simulink model "KFFA_LADRC_Quadrotor"  (R2026a)
settings: Solver=ode1  StopTime=15.0  FixedStep=0.001
InitFcn:
  | setup;
undefined symbols (not defined in the file or in its folder): b0_z, g, Ix, Iy, Iz, Kf, l0, M, Q_kf, R_kf, wc_z, wo_z, z2
settings Model: Creator=thanu  LastModifiedBy=thanu
settings DebuggingCC: UnderSpecifiedDimensionMsg=warning

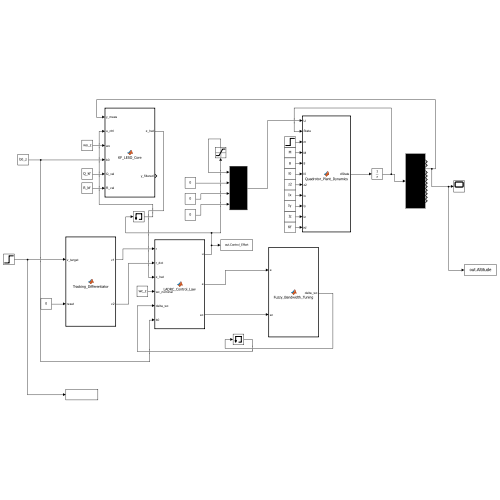
[thumbnail: Simulink's stored preview of the top-level diagram]
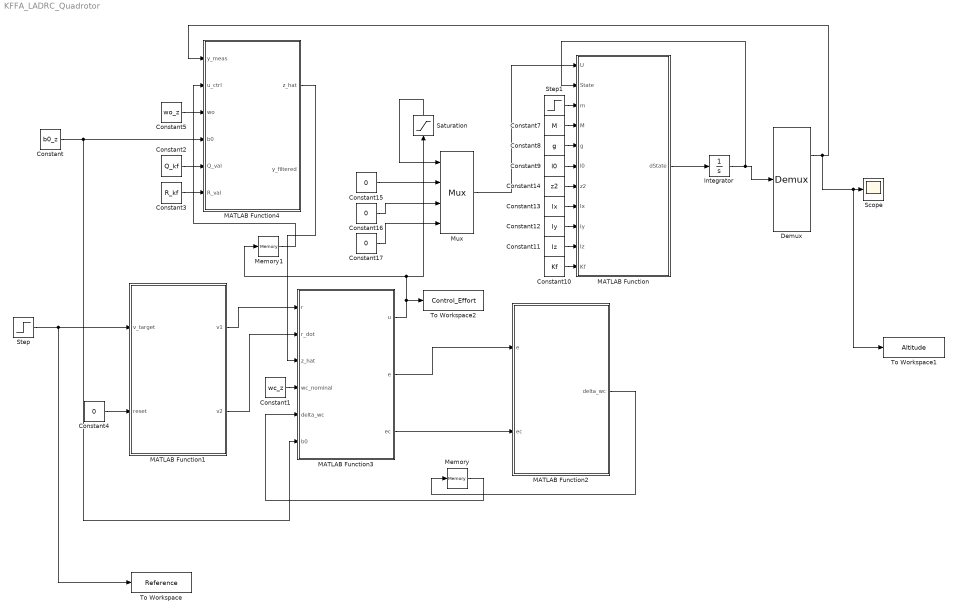
== system KFFA_LADRC_Quadrotor ==
  Constant : Constant  Value=b0_z
  Constant1 : Constant  Value=wc_z
  Constant10 : Constant  Value=Kf
  Constant11 : Constant  Value=Iz
  Constant12 : Constant  Value=Iy
  Constant13 : Constant  Value=Ix
  Constant14 : Constant  Value=z2
  Constant{4,15..17} (4 alike) : Constant  Value=0
  Constant2 : Constant  Value=Q_kf
  Constant3 : Constant  Value=R_kf
  Constant5 : Constant  Value=wo_z
  Constant7 : Constant  Value=M
  Constant8 : Constant  Value=g
  Constant9 : Constant  Value=l0
  Demux : Demux  Outputs=12
  Integrator : Integrator  InitialCondition=zeros(12,1)
  MATLAB Function : MATLAB Function  TreatAsAtomicUnit=on
  MATLAB Function1 : MATLAB Function  TreatAsAtomicUnit=on
  MATLAB Function2 : MATLAB Function  TreatAsAtomicUnit=on
  MATLAB Function3 : MATLAB Function  TreatAsAtomicUnit=on
  MATLAB Function4 : MATLAB Function  TreatAsAtomicUnit=on
  Memory : Memory
  Memory1 : Memory
  Mux : Mux
  Saturation : Saturate  UpperLimit=650  LowerLimit=0
  Scope : Scope
      settings: ActiveDisplayYMinimum=3.8784295191578879  ActiveDisplayYMaximum=5.8241533888840671
  Step : Step  FinalValue=5  SampleTime=0
  Step1 : Step  Time=5  FinalValue=m_payload_val  SampleTime=0
  To Workspace : ToWorkspace  VariableName=Reference  SampleTime=-1
  To Workspace1 : ToWorkspace  VariableName=Altitude  SampleTime=-1
  To Workspace2 : ToWorkspace  VariableName=Control_Effort  SampleTime=-1
  wires:
  Step/1 -> To Workspace/1, MATLAB Function1/1(v_target)
  Constant4/1 -> MATLAB Function1/2(reset)
  MATLAB Function1/1(v1) -> MATLAB Function3/1(r)
  MATLAB Function1/2(v2) -> MATLAB Function3/2(r_dot)
  MATLAB Function3/2(e) -> MATLAB Function2/1(e)
  MATLAB Function3/3(ec) -> MATLAB Function2/2(ec)
  MATLAB Function4/1(z_hat) -> MATLAB Function3/3(z_hat)
  Mux/1 -> MATLAB Function/1(U)
  MATLAB Function/1(dState) -> Integrator/1
  Integrator/1 -> Demux/1, MATLAB Function/2(State)
  Demux/3 -> To Workspace1/1, Scope/1, MATLAB Function4/1(y_meas)
  Constant1/1 -> MATLAB Function3/4(wc_nominal)
  Constant3/1 -> MATLAB Function4/6(R_val)
  Constant2/1 -> MATLAB Function4/5(Q_val)
  Step1/1 -> MATLAB Function/3(m)
  Constant7/1 -> MATLAB Function/4(M)
  Constant8/1 -> MATLAB Function/5(g)
  Constant9/1 -> MATLAB Function/6(l0)
  Constant10/1 -> MATLAB Function/11(Kf)
  Constant11/1 -> MATLAB Function/10(Iz)
  Constant12/1 -> MATLAB Function/9(Iy)
  Constant13/1 -> MATLAB Function/8(Ix)
  Constant14/1 -> MATLAB Function/7(z2)
  Constant15/1 -> Mux/2
  Constant16/1 -> Mux/3
  Constant17/1 -> Mux/4
  Constant/1 -> MATLAB Function3/6(b0), MATLAB Function4/4(b0)
  Constant5/1 -> MATLAB Function4/3(wo)
  MATLAB Function2/1(delta_wc) -> Memory/1
  Memory/1 -> MATLAB Function3/5(delta_wc)
  Memory1/1 -> MATLAB Function4/2(u_ctrl)
  MATLAB Function3/1(u) -> To Workspace2/1, Memory1/1, Saturation/1
  Saturation/1 -> Mux/1

== matlab function KFFA_LADRC_Quadrotor/MATLAB Function1 ==
  settings: updateMethod=DISCRETE
  data: v_target input; v1 output; reset input; v2 output
function [v1, v2] = Tracking_Differentiator(v_target, reset)
    % Discrete state retention
    persistent x1 x2
    if isempty(x1) || reset > 0.5
        x1 = 0;
        x2 = 0;
    end

    h  = 0.001;   % Integration step size
    h0 = 0.1;     % Smoothing factor
    r  = 20;     % Velocity factor

    % fhan algorithm (Eq. 16)
    x_err = x1 - v_target;
    d  = r * h0;
    d0 = h0 * d;
    y  = x_err + h0 * x2;
    a0 = sqrt(d^2 + 8 * r * abs(y));
    
    if abs(y) <= d0
        a = x2 + y / h0;
    else
        a = x2 + 0.5 * (a0 - d) * sign(y);
    end

    if abs(a) <= d
        fhan_val = -r * a / d;
    else
        fhan_val = -r * sign(a);
    end

    % Transition state update (Eq. 17)
    x1 = x1 + h * x2;
    x2 = x2 + h * fhan_val;

    v1 = x1;  % Smoothed reference
    v2 = x2;  % Smoothed derivative of reference
end

== matlab function KFFA_LADRC_Quadrotor/MATLAB Function ==
  data: U input; dState output; State input; m input; M input; g input; l0 input; z2 input; Ix input; Iy input; Iz input; Kf input
function dState = Quadrotor_Plant_Dynamics(U, State, m, M, g, l0, z2, Ix, Iy, Iz, Kf)
    x_dot     = State(4);
    y_dot     = State(5);
    z_dot     = State(6);
    xi        = State(7);
    delta     = State(8);
    eta       = State(9);
    xi_dot    = State(10);
    delta_dot = State(11);
    eta_dot   = State(12);

    U1 = U(1);  % Total lift force (N)
    U2 = U(2);  % Roll torque
    U3 = U(3);  % Pitch torque
    U4 = U(4);  % Yaw torque

    m_total = M + m;

    % Position Dynamics
    x_ddot = (U1 * (cos(xi)*sin(delta)*cos(eta) + sin(xi)*sin(eta)) - Kf * x_dot) / m_total;
    y_ddot = (U1 * (cos(xi)*sin(delta)*sin(eta) - sin(xi)*cos(eta)) - Kf * y_dot) / m_total;
    z_ddot = (U1 * cos(xi) * cos(delta) - Kf * z_dot) / m_total - g;

    % Attitude Dynamics
    xi_ddot    = (U2 * l0 + (Iz - Iy) * delta_dot * eta_dot - l0 * Kf * xi_dot) / Ix;
    delta_ddot = (U3 * l0 + (Ix - Iz) * xi_dot * eta_dot - l0 * Kf * delta_dot) / Iy;
    eta_ddot   = (U4 + (Iy - Ix) * xi_dot * delta_dot - Kf * eta_dot) / Iz;

    dState = [x_dot; y_dot; z_dot; x_ddot; y_ddot; z_ddot; ...
              xi_dot; delta_dot; eta_dot; xi_ddot; delta_ddot; eta_ddot];
end

== matlab function KFFA_LADRC_Quadrotor/MATLAB Function2 ==
  data: e input; delta_wc output; ec input
function delta_wc = Fuzzy_Bandwidth_Tuning(e, ec)
    % Domain mapping: saturate inputs to [-4, 4]
    e_val  = max(-4, min(4, e));
    ec_val = max(-4, min(4, ec));

    % 7 Triangular Membership Functions:
    % Centers: [-4, -2.67, -1.33, 0, 1.33, 2.67, 4]
    centers = [-4, -2.67, -1.33, 0, 1.33, 2.67, 4];
    
    mu_e  = zeros(1, 7);
    mu_ec = zeros(1, 7);
    for k = 1:7
        c = centers(k);
        width = 1.33;
        mu_e(k)  = max(0, 1 - abs(e_val - c)/width);
        mu_ec(k) = max(0, 1 - abs(ec_val - c)/width);
    end

    % Rule Table 2 Output Centers (-4 to +4)
    % NB=-4, NM=-2.67, NS=-1.33, ZO=0, PS=1.33, PM=2.67, PB=4
    NB = -4; NM = -2.67; NS = -1.33; ZO = 0; PS = 1.33; PM = 2.67; PB = 4;

    % 7x7 Rule Matrix from Table 2 of Paper:
    Rule_Table = [ ...
        PB, PB, PB, PB, PS, ZO, ZO; ... % NB
        PB, PB, PM, PM, PS, ZO, ZO; ... % NM
        PM, PM, PS, PS, ZO, ZO, NS; ... % NS
        PM, PS, PS, ZO, NS, NS, NM; ... % ZO
        PS, ZO, ZO, NS, NM, NM, NM; ... % PS
        ZO, ZO, NS, NM, NM, NB, NB; ... % PM
        ZO, NS, NM, NM, NB, NB, NB  ... % PB
    ];

    % Defuzzification (Weighted Average / Centroid, Eq. 40)
    num = 0;
    den = 0;
    for i = 1:7
        for j = 1:7
            weight = mu_e(i) * mu_ec(j);
            num = num + weight * Rule_Table(i, j);
            den = den + weight;
        end
    end

    if den == 0
        delta_wc = 0;
    else
        delta_wc = num / den;
    end
end

== matlab function KFFA_LADRC_Quadrotor/MATLAB Function3 ==
  data: r input; u output double size=[1 1]; r_dot input; z_hat input; wc_nominal input; delta_wc input; b0 input; e output double size=[1 1]; ec output double size=[1 1]
function [u, e, ec] = LADRC_Control_Law(r, r_dot, z_hat, wc_nominal, delta_wc, b0)
    z1 = z_hat(1);
    z2 = z_hat(2);
    z3 = z_hat(3); % Estimated disturbance (contains -g and drag)

    % Tracking errors (Target - Estimated)
    e  = r(1) - z1;
    ec = r_dot(1) - z2;

    % Controller bandwidth
    wc = max(2.0, wc_nominal(1) + delta_wc(1));
    kp = wc^2;
    kd = 2 * wc;

    % PD tracking law
    u0 = kp * e + kd * ec;

    % Disturbance rejection: u = (u0 - f) / b0
    % Since gravity creates negative acceleration, z3 is negative, so -z3 adds positive thrust
    u_raw = (u0 - z3) / b0(1);

    % Physical quadrotor motor saturation (0 N to 350 N)
    u = max(0.0, min(650.0, u_raw));
end

== matlab function KFFA_LADRC_Quadrotor/MATLAB Function4 ==
  settings: updateMethod=DISCRETE
  data: y_meas input; z_hat output; u_ctrl input; wo input; b0 input; Q_val input; R_val input; y_filtered output
function [z_hat, y_filtered] = KF_LESO_Core(y_meas, u_ctrl, wo, b0, Q_val, R_val)
    persistent z1 z2 z3 y_f
    dt = 0.001;

    if isempty(z1)
        z1 = 0;
        z2 = 0;
        z3 = -9.8;  
        y_f = 0;
    end

   
    alpha = 0.85; 
    y_f = alpha * y_f + (1 - alpha) * y_meas(1);
    y_filtered = y_f;

    wo_val = wo(1);
    beta1 = 3 * wo_val;
    beta2 = 3 * (wo_val^2);
    beta3 = wo_val^3;

    e_obs = z1 - y_filtered;

    dz1 = z2 - beta1 * e_obs;
    dz2 = z3 - beta2 * e_obs + b0(1) * u_ctrl(1);
    dz3 = -beta3 * e_obs;

    z1 = z1 + dz1 * dt;
    z2 = z2 + dz2 * dt;
    z3 = z3 + dz3 * dt;

    z3 = max(-80.0, min(80.0, z3));

    z_hat = [z1; z2; z3];
end
